simulink model "usv_dynamics"  (R2026b)
settings: Solver=VariableStepAuto  StopTime=30
settings Model: Creator=pablo  LastModifiedBy=pablo

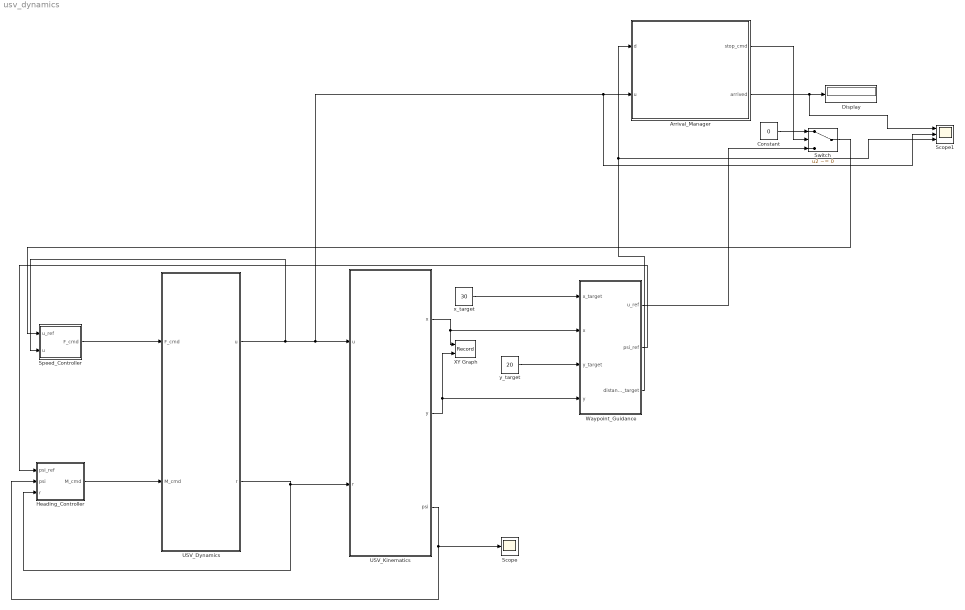
== system usv_dynamics ==
  Arrival_Manager : Stateflow chart  TreatAsAtomicUnit=on
  Constant : Constant  Value=0
  Display : Display
  Heading_Controller : Subsystem
  Scope : Scope
      settings: ActiveDisplayYMinimum=-0.087499307592752887  ActiveDisplayYMaximum=0.78749376833477613
  Scope1 : Scope  NumInputPorts=3
      settings: ActiveDisplayYMinimum=1.2212398888470908  ActiveDisplayYMaximum=35.982660289446031
  Speed_Controller : Subsystem
  Switch : Switch  Criteria=u2 ~= 0  SaturateOnIntegerOverflow=off  InputSameDT=off
  USV_Dynamics : Subsystem
  USV_Kinematics : Subsystem
  Waypoint_Guidance : Subsystem
  XY Graph : Record  NumPorts=2.0  FileSettingsInternal="{\"entries\":[{\"content\":{\"excelSettings\":{\"content\":{},\"type\":\"Streamout.ExcelSettings\"},\"parquetSettings\":{\"content\":{},\"type\":\"Streamout.ParquetSettings\"}},\"type\":\"Streamout.FileSettingStorage\",\"uuid\":\"\"}],\"packageUris\":[\"http:\\/\\/schema.mathworks.com\\/mf0\\/streamout_blocks\\/R2020a\"],\"version\":\"1.0\"}"  FrameSettings=[0, 0]  Layout=[1 1]  SignalsInternal="{\"entries\":[{\"content\":{\"signals\":[{\"content\":{\"blockPath\":[],\"dimensions\":[1],\"domain\":\"\",\"lineColor\":\"#a2142f\",\"plots\":[ 1 ],\"port\":1,\"sid\":[\"\"],\"signalID\":1,\"signalName\":\"USV_Kinematics:1\"},\"type\":\"RecordBlkView.Signal\",\"uuid\":\"\"},{\"content\":{\"blockPath\":[],\"dimensions\":[1],\"domain\":\"\",\"lineColor\":\"#139fff\",\"plots\":[ 1 ],\"port\":2,\"sid\":[\"\"],\"signalID\":2,\"signalName\":\"USV_Kinematics:2\"},\"type\":\"RecordBlkView.Signal\",\"uuid\":\"\"}]},\"type\":\"RecordBlkView.InputSignals\",\"uuid\":\"\"}],\"packageUris\":[\"http:\\/\\/schema.mathworks.com\\/mf0\\/streamout_blocks\\/R2020a\"],\"version\":\"1.0\"}"  VisualizationBindings="{\"xyplotplugin\":{\"info\":[{\"series\":[{\"bindingParametersList\":[{\"parameter\":\"X-Axis\",\"signalID\":1,\"signalName\":\"USV_Kinematics:1\"},{\"parameter\":\"Y-Axis\",\"signalID\":2,\"signalName\":\"USV_Kinematics:2\"}],\"seriesID\":0}],\"subplotID\":1}]}}"  CompatibilityTag=XY
  x_target : Constant  Value=30
  y_target : Constant  Value=20
  wires:
  USV_Dynamics/1(u) -> Speed_Controller/2(u), Scope1/2, Arrival_Manager/2(u), USV_Kinematics/1(u)
  USV_Dynamics/2(r) -> USV_Kinematics/2(r), Heading_Controller/3(r)
  Speed_Controller/1(F_cmd) -> USV_Dynamics/1(F_cmd)
  Heading_Controller/1(M_cmd) -> USV_Dynamics/2(M_cmd)
  USV_Kinematics/3(psi) -> Scope/1, Heading_Controller/2(psi)
  USV_Kinematics/1(x) -> XY Graph/1, Waypoint_Guidance/2(x)
  USV_Kinematics/2(y) -> XY Graph/2, Waypoint_Guidance/4(y)
  x_target/1 -> Waypoint_Guidance/1(x_target)
  y_target/1 -> Waypoint_Guidance/3(y_target)
  Waypoint_Guidance/2(psi_ref) -> Heading_Controller/1(psi_ref)
  Waypoint_Guidance/1(u_ref) -> Switch/3
  Arrival_Manager/1(stop_cmd) -> Switch/2
  Constant/1 -> Switch/1
  Switch/1 -> Speed_Controller/1(u_ref)
  Arrival_Manager/2(arrived) -> Scope1/1, Display/1
  Waypoint_Guidance/3(distance_to_target) -> Arrival_Manager/1(d), Scope1/3

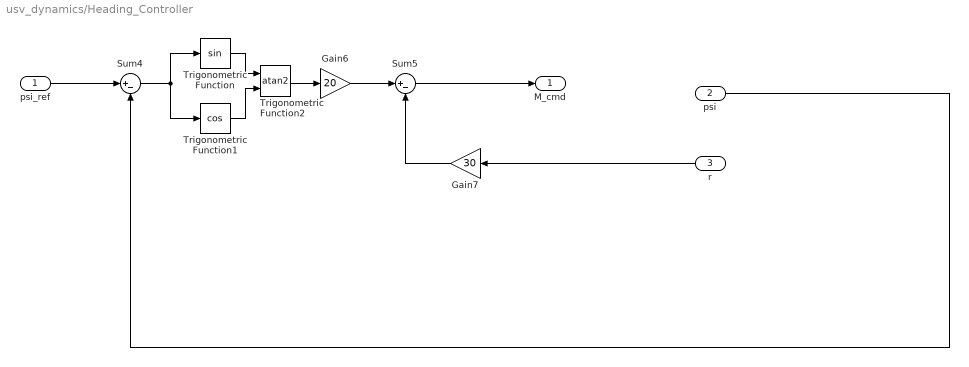
== system usv_dynamics/Heading_Controller ==
  psi_ref : Inport
  psi : Inport  Port=2
  r : Inport  Port=3
  Gain6 : Gain  Gain=20
  Gain7 : Gain  Gain=30
  Sum4 : Sum  Inputs=|+-
  Sum5 : Sum  Inputs=|+-
  Trigonometric Function : Trigonometry
  Trigonometric Function1 : Trigonometry  Operator=cos
  Trigonometric Function2 : Trigonometry  Operator=atan2
  M_cmd : Outport
  wires:
  Sum5/1 -> M_cmd/1
  psi_ref/1 -> Sum4/1
  r/1 -> Gain7/1
  Gain6/1 -> Sum5/1
  psi/1 -> Sum4/2
  Gain7/1 -> Sum5/2
  Sum4/1 -> Trigonometric Function/1, Trigonometric Function1/1
  Trigonometric Function/1 -> Trigonometric Function2/1
  Trigonometric Function1/1 -> Trigonometric Function2/2
  Trigonometric Function2/1 -> Gain6/1

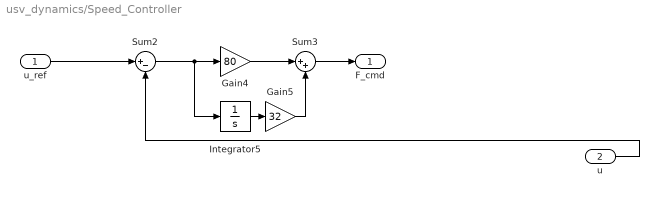
== system usv_dynamics/Speed_Controller ==
  u_ref : Inport
  u : Inport  Port=2
  Gain4 : Gain  Gain=80
  Gain5 : Gain  Gain=32
  Integrator5 : Integrator
  Sum2 : Sum  Inputs=|+-
  Sum3 : Sum  Inputs=|++
  F_cmd : Outport
  wires:
  Integrator5/1 -> Gain5/1
  u_ref/1 -> Sum2/1
  u/1 -> Sum2/2
  Gain5/1 -> Sum3/2
  Sum2/1 -> Integrator5/1, Gain4/1
  Gain4/1 -> Sum3/1
  Sum3/1 -> F_cmd/1

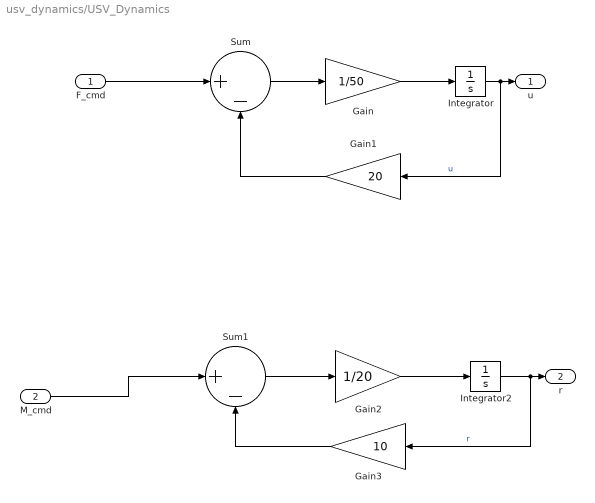
== system usv_dynamics/USV_Dynamics ==
  F_cmd : Inport
  M_cmd : Inport  Port=2
  Gain : Gain  Gain=1/50
  Gain1 : Gain  Gain=20
  Gain2 : Gain  Gain=1/20
  Gain3 : Gain  Gain=10
  Integrator : Integrator
  Integrator2 : Integrator
  Sum : Sum  Inputs=|+-
  Sum1 : Sum  Inputs=|+-
  u : Outport
  r : Outport  Port=2
  wires:
  F_cmd/1 -> Sum/1
  Gain2/1 -> Integrator2/1
  Gain3/1 -> Sum1/2
  Integrator/1 -> Gain1/1, u/1  "u"
  Sum/1 -> Gain/1
  Gain/1 -> Integrator/1
  Gain1/1 -> Sum/2
  Sum1/1 -> Gain2/1
  Integrator2/1 -> Gain3/1, r/1  "r"
  M_cmd/1 -> Sum1/1

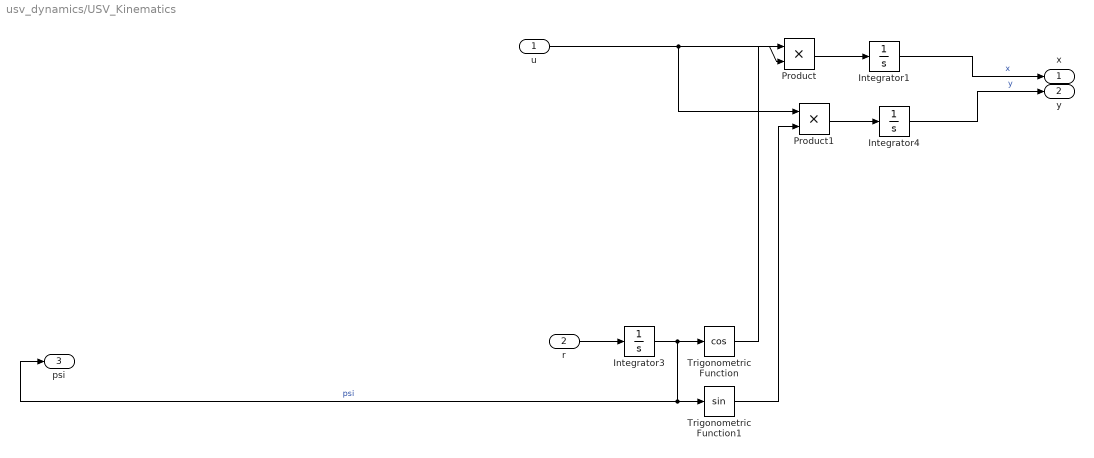
== system usv_dynamics/USV_Kinematics ==
  u : Inport
  r : Inport  Port=2
  Integrator1 : Integrator
  Integrator3 : Integrator
  Integrator4 : Integrator
  Product : Product
  Product1 : Product
  Trigonometric Function : Trigonometry  Operator=cos
  Trigonometric Function1 : Trigonometry
  x : Outport
  y : Outport  Port=2
  psi : Outport  Port=3
  wires:
  Integrator3/1 -> psi/1, Trigonometric Function1/1, Trigonometric Function/1  "psi"
  Trigonometric Function/1 -> Product/1
  u/1 -> Product1/1, Product/2
  Product/1 -> Integrator1/1
  Product1/1 -> Integrator4/1
  r/1 -> Integrator3/1
  Trigonometric Function1/1 -> Product1/2
  Integrator1/1 -> x/1  "x"
  Integrator4/1 -> y/1  "y"

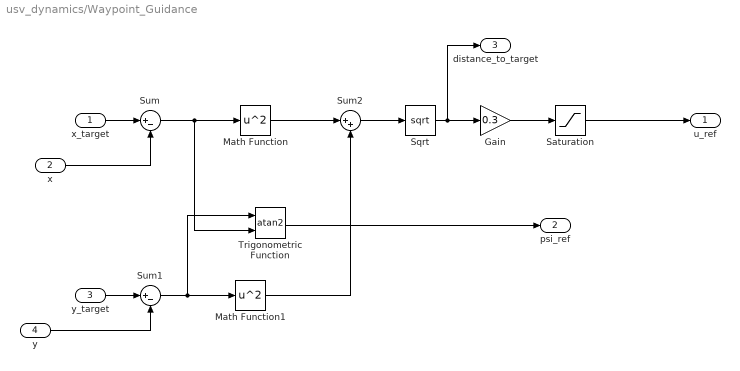
== system usv_dynamics/Waypoint_Guidance ==
  x_target : Inport
  x : Inport  Port=2
  y_target : Inport  Port=3
  y : Inport  Port=4
  Gain : Gain  Gain=0.3
  Math Function : Math  Operator=square
  Math Function1 : Math  Operator=square
  Saturation : Saturate  UpperLimit=3  LowerLimit=0
  Sqrt : Sqrt
  Sum : Sum  Inputs=|+-
  Sum1 : Sum  Inputs=|+-
  Sum2 : Sum  Inputs=|++
  Trigonometric Function : Trigonometry  Operator=atan2
  u_ref : Outport
  psi_ref : Outport  Port=2
  distance_to_target : Outport  Port=3
  wires:
  Math Function/1 -> Sum2/1
  Sum/1 -> Trigonometric Function/2, Math Function/1
  Gain/1 -> Saturation/1
  Sqrt/1 -> distance_to_target/1, Gain/1
  Sum1/1 -> Trigonometric Function/1, Math Function1/1
  Math Function1/1 -> Sum2/2
  Sum2/1 -> Sqrt/1
  Trigonometric Function/1 -> psi_ref/1
  x_target/1 -> Sum/1
  Saturation/1 -> u_ref/1
  x/1 -> Sum/2
  y_target/1 -> Sum1/1
  y/1 -> Sum1/2

== stateflow chart usv_dynamics/Arrival_Manager ==
  state Navigating
    entry:
    stop_cmd = 0;
    arrived = 0;
  state Braking
    entry:
    stop_cmd = 1;
    arrived = 0;
  state Arrived
    entry:
    stop_cmd = 1;
    arrived = 1;
  (default) -> Navigating
  Navigating -> Braking : [d <= 0.5]
  Braking -> Arrived : [d <= 0.5 && abs(u) <= 0.05]
  data: d input; u input; stop_cmd output; arrived output
